simulink model "sm_StabilityStudy"  (R2020b)
settings: Solver=VariableStepAuto  StartTime=0.0  StopTime=2000  RelTol=1e-3
values from neighbouring files (symbols this model uses):
  ACCEPTABLE_DELTA = 0.05    [code_DDPG_Training.m]    (also in code_Experimental_Setup.m; code_SA_TF_Estimator.m)
  TF_ClosedLoop_TD = feedback(tf_Plant_TD*tf_Controller, 1)    [code_SA_TF_Estimator.m]
  TIME_DELAY = 2.5/2    (= 1.25)    [code_DDPG_Training.m]    (also in code_Experimental_Setup.m; code_SA_TF_Estimator.m = 2.5)
  Ts = 1.0    (= 1)    [code_DDPG_Training.m]    (also in code_Experimental_Setup.m; code_SA_TF_Estimator.m)
undefined symbols (not defined in the file or in its folder): DiscIntNeverNeededParam, sigbuilder_block
libraries: simulink x2, rllib x1
settings Model: Creator=rajeshs  LastModifiedBy=rajeshs
settings SFSimCC: CustomCodeUndefinedFunction=UseInterfaceOnly

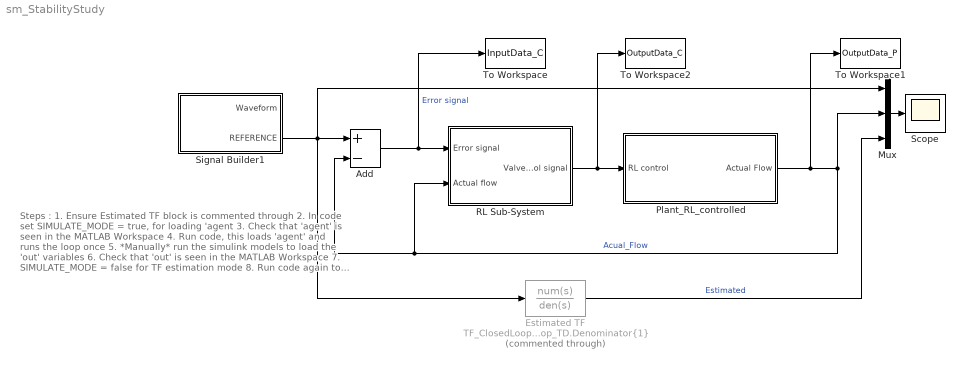
== system sm_StabilityStudy ==
  note: Steps :
      | 1. Ensure Estimated TF block is commented through
      | 2. In code set SIMULATE_MODE = true, for loading 'agent
      | 3. Check that 'agent' is seen in the MATLAB Workspace
      | 4. Run code, this loads 'agent' and runs the loop once
      | 5. *Manually* run the simulink models to load the 'out' variables
      | 6. Check that 'out' is seen in the MATLAB Workspace
      | 7. SIMULATE_MODE = false for TF estimation mode
      | 8. Run code again to estimate TFs
  Add : Sum  Inputs=+-
  Estimated TF : TransferFcn  Commented=through  Numerator=TF_ClosedLoop_TD.Numerator{1}  Denominator=TF_ClosedLoop_TD.Denominator{1}
  Mux : Mux  Inputs=3
  Plant_RL_controlled : Subsystem
  RL Sub-System : Subsystem
  Scope : Scope
  Signal Builder1 : Subsystem  Tag=STV Subsys  LoadFcn=sigbuilder_block('load');  StartFcn=sigbuilder_block('start');  StopFcn=sigbuilder_block('stop');  ClipboardFcn=sigbuilder_block('clipboard');  mask(Sigbuilder block){tuvar=[0:10]}
      mask help: Simulink:masks:SigbuilderBlock_MD
      mask init:
      | if ~strcmp(get_param(bdroot(gcbh),'SimulationStatus'),'stopped') tuvar = sigbuilder_block('maskInit'); end
      settings: CopyFcn=sigbuilder_block('copy');  DeleteFcn=sigbuilder_block('delete');  ModelCloseFcn=sigbuilder_block('modelClose');  PreSaveFcn=sigbuilder_block('preSave');  PauseFcn=sigbuilder_block('pause');  ContinueFcn=sigbuilder_block('continue');  NameChangeFcn=sigbuilder_block('namechange');  OpenFcn=sigbuilder_block('open',[12.75 50.25 1005.75 462 ]);  CloseFcn=sigbuilder_block('close');
      mask Display: plot(0, 0, 100, 100,[2, 2, 32, 32, 2], [68, 8, 8, 68, 68],[32, 2], [38, 38], [32, 19, 2],[53, 60, 44], [32, 17, 17, 2],[16, 16, 31, 31]);txt = getActiveGroup(gcbh);text(2, 100, txt,'verticalAlignment', 'top');
  To Workspace : ToWorkspace  VariableName=InputData_C  SaveFormat=Timeseries  SampleTime=-1
  To Workspace1 : ToWorkspace  VariableName=OutputData_P  SaveFormat=Timeseries  SampleTime=-1
  To Workspace2 : ToWorkspace  VariableName=OutputData_C  SaveFormat=Timeseries  SampleTime=-1
  wires:
  Mux/1 -> Scope/1
  Add/1 -> RL Sub-System/1(Error signal), To Workspace/1  "Error signal"
  Plant_RL_controlled/1(Actual Flow) -> To Workspace1/1, Mux/2, RL Sub-System/2(Actual flow), Add/2  "Acual_Flow"
  Signal Builder1/2(REFERENCE) -> Estimated TF/1, Mux/1, Add/1
  RL Sub-System/1(Valve control signal) -> Plant_RL_controlled/1(RL control), To Workspace2/1
  Estimated TF/1 -> Mux/3  "Estimated"

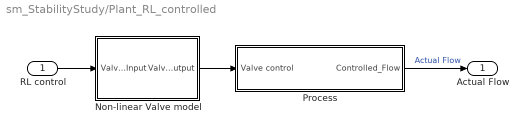
== system sm_StabilityStudy/Plant_RL_controlled ==
  RL control : Inport
  Non-linear Valve model : Subsystem
  Process : Subsystem
  Actual Flow : Outport  VectorParamsAs1DForOutWhenUnconnected=off
  wires:
  Non-linear Valve model/1(ValveOutput) -> Process/1(Valve control)
  Process/1(Controlled_Flow) -> Actual Flow/1  "Actual Flow"
  RL control/1 -> Non-linear Valve model/1(ValveInput)

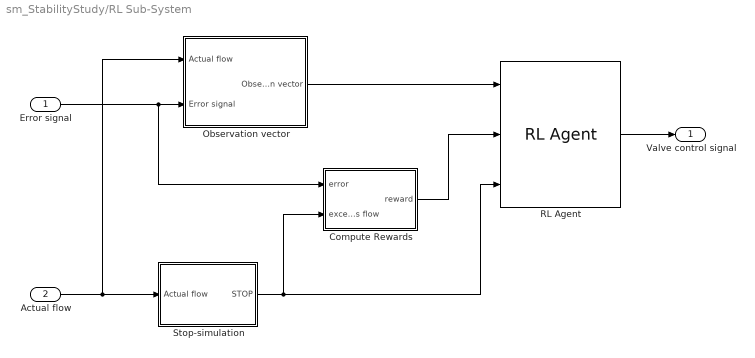
== system sm_StabilityStudy/RL Sub-System ==
  Error signal : Inport
  Actual flow : Inport  Port=2
  Compute Rewards : Subsystem
  Observation vector : Subsystem
  RL Agent : rllib/RL Agent  Agent=agent  ProvideReward=on  ProvideIsDone=on  ProvideCumRwd=off  TreatAsDirectFeedthrough=on  CollectLoggedSignals=on  CollectModelStates=on
  Stop-simulation : Subsystem
  Valve control signal : Outport  VectorParamsAs1DForOutWhenUnconnected=off
  wires:
  Stop-simulation/1(STOP) -> RL Agent/3, Compute Rewards/2(exceeds flow)
  Error signal/1 -> Compute Rewards/1(error), Observation vector/2(Error signal)
  Compute Rewards/1(reward) -> RL Agent/2
  Observation vector/1(Observation vector) -> RL Agent/1
  RL Agent/1 -> Valve control signal/1
  Actual flow/1 -> Observation vector/1(Actual flow), Stop-simulation/1(Actual flow)

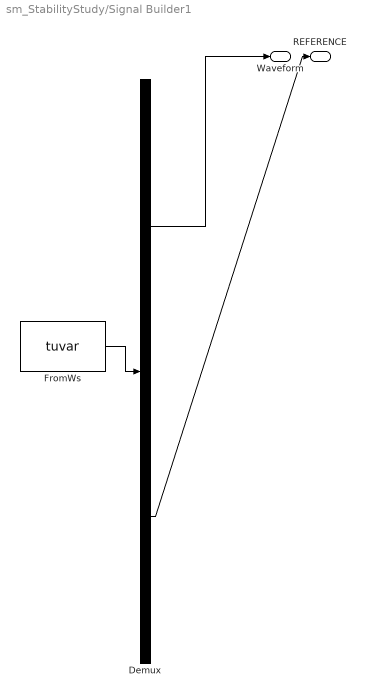
== system sm_StabilityStudy/Signal Builder1 ==
  Demux : Demux  Tag=STV Demux  Outputs=2
      settings: DisplayOption=none
  FromWs : FromWorkspace  Tag=STV FromWs  VariableName=tuvar
      SigBuilderData=|
      | common.afterFinalStr = 'Extrapolate'
      | common.sampleTime = 0
      | dataSet.timeRange = [0 2000]
      | dataSet.name = 'Signals'
      | sbobj.Groups.Name = 'Signals'
      | sbobj.Groups.Signals(1).Name = 'Waveform'
      | sbobj.Groups.Signals(1).XData = [0 752 752 1500 1500 1750 1750 2000]
      | sbobj.Groups.Signals(1).YData = [10 10 2.5 2.5 7.5 7.5 2.5 2.5]
      | sbobj.Groups.Signals(2).Name = 'REFERENCE'
      | sbobj.Groups.Signals(2).XData = [0 2000]
      | sbobj.Groups.Signals(2).YData = [100 100]
      | sbobj.Groups.TimeRange = [0 2000]
  Waveform : Outport  Tag=STV Outport  VectorParamsAs1DForOutWhenUnconnected=off
  REFERENCE : Outport  Tag=STV Outport  Port=2  VectorParamsAs1DForOutWhenUnconnected=off
  wires:
  Demux/1 -> Waveform/1
  FromWs/1 -> Demux/1
  Demux/2 -> REFERENCE/1

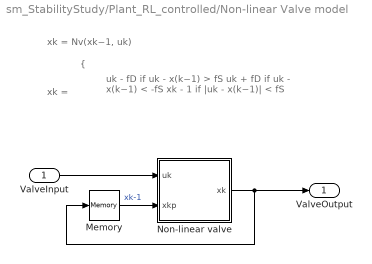
== system sm_StabilityStudy/Plant_RL_controlled/Non-linear Valve model ==
  note: xk = Nv(xk−1, uk)
  note: {
  note: xk =
  note: uk - fD if uk - x(k−1) > fS
      | uk + fD if uk - x(k−1) < -fS
      | xk - 1 if |uk - x(k−1)| < fS
  ValveInput : Inport
  Memory : Memory
  Non-linear valve : MATLAB Function  TreatAsAtomicUnit=on
  ValveOutput : Outport  VectorParamsAs1DForOutWhenUnconnected=off
  wires:
  Non-linear valve/1(xk) -> ValveOutput/1, Memory/1
  Memory/1 -> Non-linear valve/2(xkp)  "xk-1"
  ValveInput/1 -> Non-linear valve/1(uk)

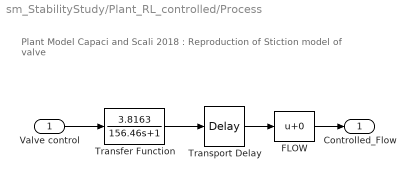
== system sm_StabilityStudy/Plant_RL_controlled/Process ==
  note: Plant Model
      |
      | Capaci and Scali 2018 : Reproduction of Stiction model of valve
  Valve control : Inport
  FLOW : Bias
  Transfer Function : TransferFcn  Numerator=[3.8163]  Denominator=[156.46 1]
  "Transport Delay " : TransportDelay  DelayTime=TIME_DELAY
  Controlled_Flow : Outport  VectorParamsAs1DForOutWhenUnconnected=off
  wires:
  FLOW/1 -> Controlled_Flow/1
  Transfer Function/1 -> "Transport Delay "/1
  Valve control/1 -> Transfer Function/1
  "Transport Delay "/1 -> FLOW/1

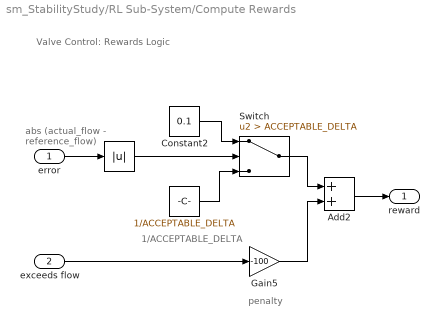
== system sm_StabilityStudy/RL Sub-System/Compute Rewards ==
  note: penalty
  note: 1/ACCEPTABLE_DELTA
  note: abs (actual_flow - reference_flow)
  note: Valve Control: Rewards Logic
  error : Inport
  exceeds flow : Inport  Port=2
  " " : Constant  Value=1/ACCEPTABLE_DELTA
  " " : Abs
  Add2 : Sum
  Constant2 : Constant  Value=0.1
  Gain5 : Gain  Gain=-100
  Switch : Switch  Criteria=u2 > Threshold  Threshold=ACCEPTABLE_DELTA
  reward : Outport  VectorParamsAs1DForOutWhenUnconnected=off
  wires:
  Gain5/1 -> Add2/2
  exceeds flow/1 -> Gain5/1
  error/1 -> " "/1
  Add2/1 -> reward/1
  " "/1 -> Switch/2
  " "/1 -> Switch/3
  Constant2/1 -> Switch/1
  Switch/1 -> Add2/1

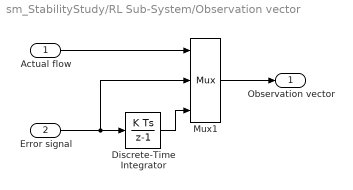
== system sm_StabilityStudy/RL Sub-System/Observation vector ==
  Actual flow : Inport
  Error signal : Inport  Port=2
  Discrete-Time Integrator : DiscreteIntegrator  SampleTime=Ts  ICPrevOutput=DiscIntNeverNeededParam  ICPrevScaledInput=DiscIntNeverNeededParam
  Mux1 : Mux  Inputs=3
  Observation vector : Outport  VectorParamsAs1DForOutWhenUnconnected=off
  wires:
  Discrete-Time Integrator/1 -> Mux1/3
  Mux1/1 -> Observation vector/1
  Error signal/1 -> Discrete-Time Integrator/1, Mux1/2
  Actual flow/1 -> Mux1/1

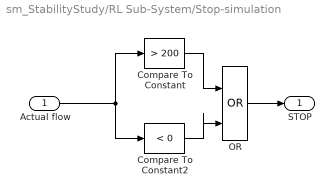
== system sm_StabilityStudy/RL Sub-System/Stop-simulation ==
  Actual flow : Inport
  Compare To Constant : simulink/Logic and Bit Operations/Compare To Constant  relop=>  const=200  OutDataTypeStr=boolean
  Compare To Constant2 : simulink/Logic and Bit Operations/Compare To Constant  relop=<  const=0  OutDataTypeStr=boolean
  OR : Logic  Operator=OR  IconShape=distinctive  AllPortsSameDT=off  OutDataTypeStr=boolean
  STOP : Outport  VectorParamsAs1DForOutWhenUnconnected=off
  wires:
  Compare To Constant/1 -> OR/1
  Actual flow/1 -> Compare To Constant/1, Compare To Constant2/1
  Compare To Constant2/1 -> OR/2
  OR/1 -> STOP/1

== matlab function sm_StabilityStudy/Plant_RL_controlled/Non-linear Valve model/Non-linear valve ==
  data: uk input; xk output; xkp input
function xk = fcn(uk, xkp)
% ----------------------------------------------------------------------------------------
% DDPG RL AGENT EVALUATION circuit Plant Model (RLVC2 | Verified 15-Jul-2020)
% Non-Linear valve model: Capaci and Scali (2018)
% Friction values conform to benchmark flow rates used in Capaci (2016)
% ----------------------------------------------------------------------------------------
% uk - fD   if uk - xk−1 > fS
% uk + fD   if uk - xk−1 < -fS
% xk - 1    if |uk - xk−1| < fS
% ----------------------------------------------------------------------------------------

    fS = 8.4;
    fD = 3.5243;
        
    t_xk = 0.0;
   
    if ((uk-xkp) > fS)
        t_xk = uk - fD;
    elseif ((uk-xkp) < -1*fS)
        t_xk = uk + fD;
    elseif (abs(uk-xkp) < fS)
        t_xk = xkp;
    end
    
xk = t_xk;
